simulink model "Pitch_Control_Hydraulic_Testrig"  (R2025a)
settings: Solver=ode15s  StartTime=0.0  StopTime=5.5  RelTol=1e-3  EnableMultiTasking=on
PostLoadFcn:
  | %open_system([bdroot '/Start Values']);
  | Pitch_Control_Hydraulic_Testrig_setparam('Initial');
  | warning off Control:analysis:ScalingIssue
  | warning off Control:transformation:StateSpaceScaling
  | warning('off','MATLAB:HandleGraphics:ObsoletedProperty:JavaFrame')
  | warning('off','physmod:common:gl:sli:rtp:InvalidNonValueReference');
undefined symbols (not defined in the file or in its folder): Actuator_Lookup, Pitch_Ki, Pitch_Kp, sigbuilder_block, WT_Params, X, Y, Z
libraries: sm_lib x6, nesl_utility x2, Hydraulic_Actuator_Lib x1, Blades_Lib x1, Pitch_System_Lib x1
Description:
  | Copyright 2009-2025 The MathWorks, Inc. MathWorks, Inc.
settings Model: Creator=smiller  LastModifiedBy=smiller
settings SolverCC: MaxConsecutiveMinStep=8  AlgebraicLoopSolver=TrustRegion
settings DataIOCC: ExternalInput=getinputstruct(op_snapshot1)  InitialState=getstatestruct(op_snapshot1)  LimitDataPoints=on  SaveFormat=Array  ReturnWorkspaceOutputs=off
settings OptimizationCC: ReuseModelBlockBuffer=off  ExpressionDepthLimit=2147483647.0  LifeSpan=inf
settings DebuggingCC: AlgebraicLoopMsg=none  UnderspecifiedInitializationDetection=Classic  MergeDetectMultiDrivingBlocksExec=none  FcnCallInpInsideContextMsg=warning  AllowSymbolicDim=off  StateNameClashWarn=warning  PregeneratedLibrarySubsystemCodeDiagnostic=none  SFUnexpectedBacktrackingDiag=warning  SFNoUnconditionalDefaultTransitionDiag=warning  SFExecutionAtInitializationDiag=none  ArithmeticOperatorsInVariantConditions=warning
settings HardwareCC: ProdBitPerPointer=32.0  ProdBitPerSizeT=32.0  ProdBitPerPtrDiffT=32.0  ProdLargestAtomicFloat=None  ProdIntDivRoundTo=Undefined  ProdEndianess=Unspecified  ProdWordSize=32.0  ProdHWDeviceType=32-bit Generic
settings ModelReferenceCC: EnableRefExpFcnMdlSchedulingChecks=on  PropagateSignalLabelsOutOfModel=off
settings SFSimCC: SimUseLocalCustomCode=off  CustomCodeUndefinedFunction=UseInterfaceOnly
settings RTWCC: RTWUseLocalCustomCode=off  GPUComputeCapability=3.5  DLArmComputeVersion=19.05
settings CodeAppCC: StateflowObjectComments=on
settings GRTTargetCC: TargetLangStandard=C89/C90 (ANSI)  CombineOutputUpdateFcns=off  GRTInterface=on
settings ConfigComp: CovMetricSettings=dw  CovSaveCumulativeToWorkspaceVar=on  CovSaveSingleToWorkspaceVar=on  CovExternalEMLEnable=off  CovSFcnEnable=off
settings SimscapeCC: SimscapeNormalizeSystem=off  SimscapeLogType=all  SimscapeLogName=simlog_Pitch_Control_Hydraulic_Testrig
settings ConfigurationSet: Description=SimMechanics 2G
settings DiagnosticsConfigSet: SimMechanicsUnconnectedFramePorts=none
settings ExplorerConfigSet: InternalSimMechanicsExplorerSettings="<ExplorerConfiguration><canonicalview>default</canonicalview><TilePanel><TileInfo><Tiles Columns=\"1\" Count=\"1\" Rows=\"1\"><Column Left=\"2\" Weight=\"1\"/><Column Left=\"651\"/><Row Top=\"2\" Weight=\"1\"/><Row Top=\"621\"/><Tile Height=\"1\" Width=\"1\" X=\"0\" Y=\"0\"/></Tiles></TileInfo><SceneInfo><SceneViewer><BGColor><R>0.80000001192092896</R><G>1</G><B>1</B></BGColor><Camera><Position><X>0.95698142051696777</X><Y>-0.28347766399383545</Y><Z>-22.851342627275898</Z></Position><Center><X>0.95698142051696777</X><Y>-0.28347766399383545</Y><Z>19.917768478393555</Z></Center><Up><X>0</X><Y>-1</Y><Z>0</Z></Up><Left>-2.3551695585250854</Left><Right>2.3551695585250854</Right><Bottom>-2.1292211294174197</Bottom><Top>2.1292211294174197</Top></Camera></SceneViewer></SceneInfo></TilePanel></ExplorerConfiguration>"

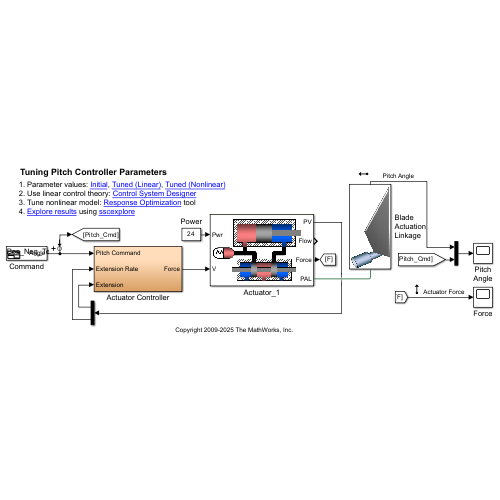
[thumbnail: Simulink's stored preview of the top-level diagram]
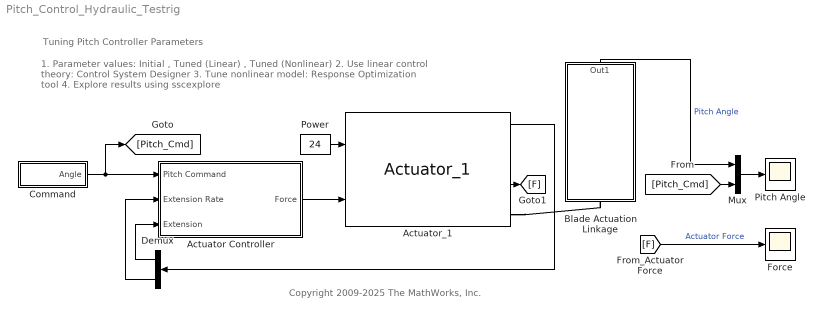
== system Pitch_Control_Hydraulic_Testrig ==
  note: Copyright 2009-2025 The MathWorks, Inc.
  note: 1. Parameter values: Initial , Tuned (Linear) , Tuned (Nonlinear)
      | 2. Use linear control theory: Control System Designer
      | 3. Tune nonlinear model: Response Optimization tool
      | 4. Explore results using sscexplore
  note: Tuning Pitch Controller Parameters
  Actuator Controller : Subsystem  AncestorBlock=Pitch_Controller_Lib/Inner Loop/Actuator Controller
      settings: LibrarySourceBlock=Pitch_Controller_Lib/Inner Loop/Actuator Controller
  Actuator_1 : Hydraulic_Actuator_Lib/Actuator_1  SystemSampleTime=-1  VariantActivationTime=update diagram  EmptyChoice=off  PassThrough=off  PassThroughVariantControl=(default)  EmptyChoiceVariantControl=(default)  AllowFlexibleInterface=on  Latency=0  AutoFrameSizeCalculation=off
  Blade Actuation Linkage : Subsystem
      mask Display: image(imread('Single_Blade_IMAGE.jpg'));
  Command : Subsystem  Tag=STV Subsys  AncestorBlock=Turbine_Input_Lib/Commands/Signal Builder  LoadFcn=sigbuilder_block('load');  StartFcn=sigbuilder_block('start');  StopFcn=sigbuilder_block('stop');  ClipboardFcn=sigbuilder_block('clipboard');  mask(Sigbuilder block){}
      mask help: Sigbuilder GUI
      mask init:
      | if ~strcmp(get_param(bdroot(gcbh),'SimulationStatus'),'stopped') tuvar = sigbuilder_block('maskInit'); end
      settings: LibrarySourceBlock=Turbine_Input_Lib/Commands/Signal Builder  CopyFcn=sigbuilder_block('copy');  DeleteFcn=sigbuilder_block('delete');  ModelCloseFcn=sigbuilder_block('modelClose');  PreSaveFcn=sigbuilder_block('preSave');  PauseFcn=sigbuilder_block('pause')  ContinueFcn=sigbuilder_block('continue')  NameChangeFcn=sigbuilder_block('namechange');  OpenFcn=sigbuilder_block('open',[214.8 226.8 550.2 360.6 ]);  CloseFcn=sigbuilder_block('close');
      mask Display: plot(0, 0, 100, 100,[2, 2, 32, 32, 2], [68, 8, 8, 68, 68],[32, 2], [38, 38], [32, 19, 2],[53, 60, 44], [32, 17, 17, 2],[16, 16, 31, 31]);txt = getActiveGroup(gcbh);text(2, 100, txt,'verticalAlignment', 'top');
  Demux : Demux  Outputs=2
  Force : Scope
      settings: ActiveDisplayYMinimum=-7000.68211  ActiveDisplayYMaximum=9615.01423  DataLoggingVariableName=Pitch_Control_H_Force_DATA
  Mux : Mux  Inputs=2
  Pitch Angle : Scope
      settings: ActiveDisplayYMinimum=-25  ActiveDisplayYMaximum=25  DataLoggingVariableName=Pitch_Control_H_Angle_DATA
  Power : Constant  Value=24
  wires:
  Blade Actuation Linkage/1(Out1) -> Mux/1  "Pitch Angle"
  Actuator Controller/1(Force) -> Actuator_1/2
  Actuator_1/1 -> Demux/1
  Demux/1 -> Actuator Controller/3(Extension)
  Demux/2 -> Actuator Controller/2(Extension Rate)
  Command/1(Angle) -> [Pitch_Cmd], Actuator Controller/1(Pitch Command)
  Mux/1 -> Pitch Angle/1
  [Pitch_Cmd] -> Mux/2
  Power/1 -> Actuator_1/1
  [F] -> Force/1  "Actuator Force"
  Actuator_1/3 -> [F]
  connections:
  Actuator_1/RConn1 -- Blade Actuation Linkage/LConn1

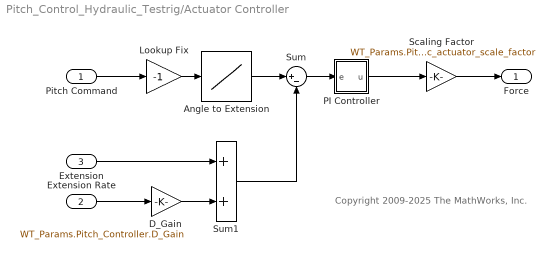
== system Pitch_Control_Hydraulic_Testrig/Actuator Controller ==
  note: Copyright 2009-2025 The MathWorks, Inc.
  Pitch Command : Inport
  Extension Rate : Inport  Port=2
  Extension : Inport  Port=3
  Angle to Extension : Lookup  InputValues=-Actuator_Lookup.angle  Table=Actuator_Lookup.extension  SaturateOnIntegerOverflow=off
  D_Gain : Gain  Gain=WT_Params.Pitch_Controller.D_Gain
  Lookup Fix : Gain  Gain=-1
  PI Controller : Subsystem
      mask Display: disp('PI')
  Scaling Factor : Gain  Gain=WT_Params.Pitch_Actuator.hydraulic_actuator_scale_factor
  Sum : Sum  Inputs=|+-
  Sum1 : Sum
  Force : Outport  VectorParamsAs1DForOutWhenUnconnected=off
  wires:
  Sum/1 -> PI Controller/1(e)
  Angle to Extension/1 -> Sum/1
  Lookup Fix/1 -> Angle to Extension/1
  D_Gain/1 -> Sum1/2
  Sum1/1 -> Sum/2
  Pitch Command/1 -> Lookup Fix/1
  Extension/1 -> Sum1/1
  PI Controller/1(u) -> Scaling Factor/1
  Extension Rate/1 -> D_Gain/1
  Scaling Factor/1 -> Force/1

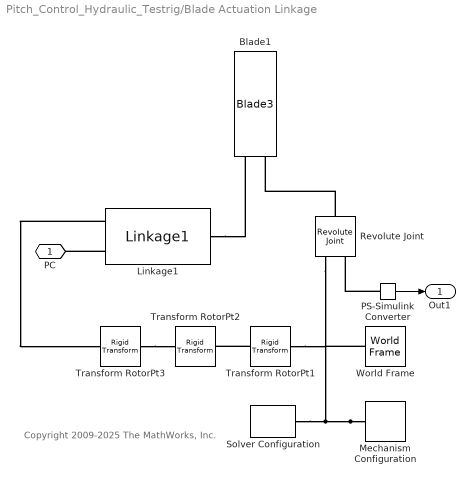
== system Pitch_Control_Hydraulic_Testrig/Blade Actuation Linkage ==
  note: Copyright 2009-2025 The MathWorks, Inc.
  Blade1 : Blades_Lib/Blades/Blade3  SystemSampleTime=-1  VariantActivationTime=update diagram  EmptyChoice=off  PassThrough=off  PassThroughVariantControl=(default)  EmptyChoiceVariantControl=(default)  AllowFlexibleInterface=on  Latency=0  AutoFrameSizeCalculation=off
  Linkage1 : Pitch_System_Lib/Hydraulic/Linkage1  SystemSampleTime=-1  VariantActivationTime=update diagram  EmptyChoice=off  PassThrough=off  PassThroughVariantControl=(default)  EmptyChoiceVariantControl=(default)  AllowFlexibleInterface=on  Latency=0  AutoFrameSizeCalculation=off
  Mechanism Configuration : sm_lib/Utilities/Mechanism Configuration  UniformGravity=Constant  GravityVector=[0 0 -9.81]*0  GravityVectorUnits=m/s^2  LinearizationDelta=0.001  JointModeTransitionNonlinearIterations=2
  PS-Simulink Converter : nesl_utility/PS-Simulink Converter  PhysicalDomain=network_engine_domain  SubClassName=ps_output  LeftPortType=input  RightPortType=output  PseudoPeriodic=off  Frequencies=[]  VectorFormat=1-D array  Unit=deg  AffineConversion=off
  Revolute Joint : sm_lib/Joints/Revolute Joint  JointMode=Normal  CompositeWrenchDir=FollowerOnBase  CompositeWrenchFrame=BaseFrame  SenseConstraintForce=off  SenseConstraintTorque=off  SenseTotalForce=off  SenseTotalTorque=off  PositionTargetSpecify=on  PositionTargetPriority=High  PositionTargetValue=0  PositionTargetValueUnits=deg  VelocityTargetSpecify=off  VelocityTargetPriority=High  VelocityTargetValue=0  VelocityTargetValueUnits=deg/s  EquilibriumPosition=0  EquilibriumPositionUnits=deg  SpringStiffness=0  SpringStiffnessUnits=N*m/deg  DampingCoefficient=WT_Params.Blade.damping  DampingCoefficientUnits=N*m/(deg/s)  LowerLimitSpecify=off  LowerLimitBound=-90  LowerLimitBoundUnits=deg  LowerLimitStiffness=1e4  LowerLimitStiffnessUnits=N*m/deg  LowerLimitDamping=10  LowerLimitDampingUnits=N*m/(deg/s)  LowerLimitTransitionRegionWidth=0.1  LowerLimitTransitionRegionWidthUnits=deg  UpperLimitSpecify=off  UpperLimitBound=90  UpperLimitBoundUnits=deg  UpperLimitStiffness=1e4  UpperLimitStiffnessUnits=N*m/deg  UpperLimitDamping=10  UpperLimitDampingUnits=N*m/(deg/s)  UpperLimitTransitionRegionWidth=0.1  UpperLimitTransitionRegionWidthUnits=deg  TorqueActuationMode=NoTorque  MotionActuationMode=ComputedMotion  SensePosition=on  SenseVelocity=off  SenseAcceleration=off  SenseTorqueForce=off  SenseLowerLimitTorqueForce=off  SenseUpperLimitTorqueForce=off
  Solver Configuration : nesl_utility/Solver Configuration  PhysicalDomain=network_engine_domain  SubClassName=solver  LeftPortType=input  RightPortType=generic  Tones=[]  Harmonics=[]  SimulateNoise=off  Profile=off  UseLocalSampling=off  EnableSwitchedLinearOptims=on  FrequencyDomain=off  UseCCode=off  RelTol=0.001  AbsTol=1e-06  MinStep=1e-09  ToWorkspace=off  RevertToSquareIcSolve=off  NumHomotopyIterations=100  PhasorMode=off  PhasorModeNumHarmonics=1  ConsistencySolver=NEWTON_FTOL  IndexReductionMethod=DerivativeReplacement  DoDC=off  ResidualTolerance=1e-9  ConsistencyTolSource=GLOBAL  ConsistencyAbsTol=0.001  ConsistencyRelTol=0.001  ConsistencyTolFactor=0.001  UseLocalSolver=off  LocalSolverChoice=NE_BACKWARD_EULER_ADVANCER  ResolveIndetEquations=on  FunctionEvalNumThread=1  LocalSolverSampleTime=.001  DoFixedCost=off  MaxNonlinIter=3  MaxModeIter=2  ComputeImpulses=off  ImpulseIterations=2  LinearAlgebra=Sparse  LinearAlgebraNumThread=0  EquationFormulation=NE_TIME_EF  DelaysMemoryBudget=1024  AutomaticFiltering=on  FilteringTimeConstant=0.001  PartitionStorageMethod=AS_NEEDED  PartitionMemoryBudget=1024  PartitionMethod=FAST  MultibodyUseLocalSolver=off  MultibodyLocalSolverChoice=ODE1  MultibodyLocalSolverSampleTime=0.001
  Transform RotorPt1 : sm_lib/Frames and Transforms/Rigid Transform  RotationMethod=None  FollAlignAxisA=+X  BaseAlignAxisA=+Y  FollAlignAxisB=+Y  BaseAlignAxisB=+Z  RotationStandardAxis=+Z  RotationAngle=0  RotationAngleUnits=deg  RotationArbitraryAxis=[0 0 1]  RotationSequenceAxes=FollowerAxes  RotationSequence=XYX  RotationSequenceAngles=[0 0 0]  RotationSequenceAnglesUnits=deg  RotationMatrix=[1 0 0; 0 1 0; 0 0 1]  Quaternion=[1 0 0 0]  TranslationMethod=Cartesian  TranslationCartesianOffset=[0 WT_Params.Blade.Actuator_Offset.z WT_Params.Blade.Actuator_Offset.y/2]  TranslationCartesianOffsetUnits=m  TranslationStandardAxis=+Z  TranslationStandardOffset=0  TranslationStandardOffsetUnits=m  TranslationROffset=0  TranslationROffsetUnits=m  TranslationThetaOffset=0  TranslationThetaOffsetUnits=deg  TranslationZOffset=0  TranslationZOffsetUnits=m
  Transform RotorPt2 : sm_lib/Frames and Transforms/Rigid Transform  RotationMethod=None  FollAlignAxisA=+X  BaseAlignAxisA=+Y  FollAlignAxisB=+Y  BaseAlignAxisB=+Z  RotationStandardAxis=+Z  RotationAngle=0  RotationAngleUnits=deg  RotationArbitraryAxis=[0 0 1]  RotationSequenceAxes=FollowerAxes  RotationSequence=XYX  RotationSequenceAngles=[0 0 0]  RotationSequenceAnglesUnits=deg  RotationMatrix=[1 0 0; 0 1 0; 0 0 1]  Quaternion=[1 0 0 0]  TranslationMethod=Cartesian  TranslationCartesianOffset=[0 0 WT_Params.Blade.Actuator_Offset.y/2]  TranslationCartesianOffsetUnits=m  TranslationStandardAxis=+Z  TranslationStandardOffset=0  TranslationStandardOffsetUnits=m  TranslationROffset=0  TranslationROffsetUnits=m  TranslationThetaOffset=0  TranslationThetaOffsetUnits=deg  TranslationZOffset=0  TranslationZOffsetUnits=m
  Transform RotorPt3 : sm_lib/Frames and Transforms/Rigid Transform  RotationMethod=StandardAxis  FollAlignAxisA=+X  BaseAlignAxisA=+Y  FollAlignAxisB=+Y  BaseAlignAxisB=+Z  RotationStandardAxis=+Y  RotationAngle=90  RotationAngleUnits=deg  RotationArbitraryAxis=[0 0 1]  RotationSequenceAxes=FollowerAxes  RotationSequence=XYX  RotationSequenceAngles=[0 0 0]  RotationSequenceAnglesUnits=deg  RotationMatrix=[1 0 0; 0 1 0; 0 0 1]  Quaternion=[1 0 0 0]  TranslationMethod=Cartesian  TranslationCartesianOffset=[WT_Params.Pitch_Actuator.cylinder_length*2 0 0]  TranslationCartesianOffsetUnits=m  TranslationStandardAxis=+Z  TranslationStandardOffset=0  TranslationStandardOffsetUnits=m  TranslationROffset=0  TranslationROffsetUnits=m  TranslationThetaOffset=0  TranslationThetaOffsetUnits=deg  TranslationZOffset=0  TranslationZOffsetUnits=m
  World Frame : sm_lib/Frames and Transforms/World Frame
  PC : PMIOPort  Side=Left
  Out1 : Outport  VectorParamsAs1DForOutWhenUnconnected=off
  wires:
  PS-Simulink Converter/1 -> Out1/1
  connections:
  Mechanism Configuration/RConn1 -- Solver Configuration/RConn1 -- World Frame/RConn1 -- Revolute Joint/RConn1 -- Transform RotorPt1/LConn1
  Transform RotorPt1/RConn1 -- Transform RotorPt2/LConn1
  Revolute Joint/LConn1 -- Blade1/LConn2
  Linkage1/LConn1 -- Blade1/LConn1
  PS-Simulink Converter/LConn1 -- Revolute Joint/RConn2
  Transform RotorPt3/LConn1 -- Transform RotorPt2/RConn1
  Linkage1/RConn1 -- Transform RotorPt3/RConn1
  Linkage1/RConn2 -- PC/RConn1

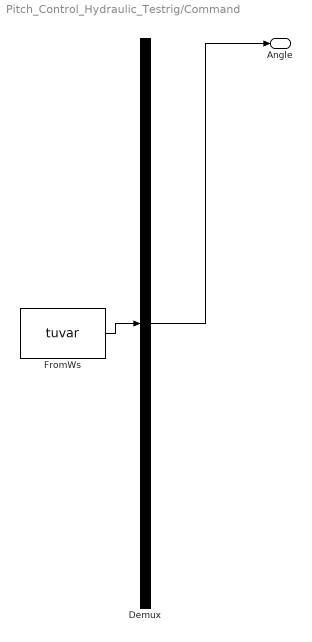
== system Pitch_Control_Hydraulic_Testrig/Command ==
  Demux : Demux  Tag=STV Demux  Outputs=1
      settings: DisplayOption=none
  FromWs : FromWorkspace  Tag=STV FromWs  VariableName=tuvar
      SigBuilderData=|
      | common.afterFinalStr = 'Extrapolate'
      | common.sampleTime = 0
      | dataSet(1).timeRange = [0 50]
      | dataSet(1).name = 'Pos_Test'
      | dataSet(2).timeRange = [0 50]
      | dataSet(2).name = 'Pos_Neg_Test'
      | dataSet(3).timeRange = [0 50]
      | dataSet(3).name = 'Step_Test'
      | sbobj.Groups(1).Name = 'Pos_Test'
      | sbobj.Groups(1).Signals.Name = 'Angle'
      | sbobj.Groups(1).Signals.XData = [0 5 5 7.5 7.5 25.1 25.1 28 28 50]
      | sbobj.Groups(1).Signals.YData = [0 0 20 20 0 0 20 20 0 0]
      | sbobj.Groups(2).Name = 'Pos_Neg_Test'
      | sbobj.Groups(2).Signals.Name = 'Angle'
      | sbobj.Groups(2).Signals.XData = [0 3 3 5.5 5.5 8 8 10.5 10.5 50]
      | sbobj.Groups(2).Signals.YData = [0 0 20 20 0 0 -20 -20 0 0]
      | sbobj.Groups(3).Name = 'Step_Test'
      | sbobj.Groups(3).Signals.Name = 'Angle'
      | sbobj.Groups(3).Signals.XData = [0 1 1 7.5 25.1 30 30 50]
      | sbobj.Groups(3).Signals.YData = [0 0 20 20 20 20 0 0]
  Angle : Outport  Tag=STV Outport  VectorParamsAs1DForOutWhenUnconnected=off
  wires:
  Demux/1 -> Angle/1
  FromWs/1 -> Demux/1

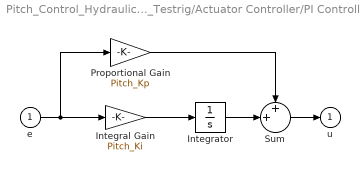
== system Pitch_Control_Hydraulic_Testrig/Actuator Controller/PI Controller ==
  e : Inport
  Integral Gain : Gain  Gain=Pitch_Ki  SaturateOnIntegerOverflow=on  OutDataTypeStr=Inherit: Same as input  ParamDataTypeStr=Inherit: Same as input
  Integrator : Integrator
  Proportional Gain : Gain  Gain=Pitch_Kp  SaturateOnIntegerOverflow=on  OutDataTypeStr=Inherit: Same as input  ParamDataTypeStr=Inherit: Same as input
  Sum : Sum  Inputs=++|  InputSameDT=on  SaturateOnIntegerOverflow=on  OutDataTypeStr=Inherit: Same as first input
  u : Outport  InitialOutput=0  VectorParamsAs1DForOutWhenUnconnected=off
  wires:
  Integral Gain/1 -> Integrator/1
  Proportional Gain/1 -> Sum/1
  Integrator/1 -> Sum/2
  e/1 -> Proportional Gain/1, Integral Gain/1
  Sum/1 -> u/1
